simulink model "mimo_2x2_zf"  (R2024b)
settings: Solver=FixedStepDiscrete  StartTime=0  StopTime=0  FixedStep=1  RelTol=1e-3
settings Model: Creator=Devansh  LastModifiedBy=Devansh
settings DataIOCC: SaveOutput=off  SignalLogging=off  SaveTime=off  ReturnWorkspaceOutputs=off

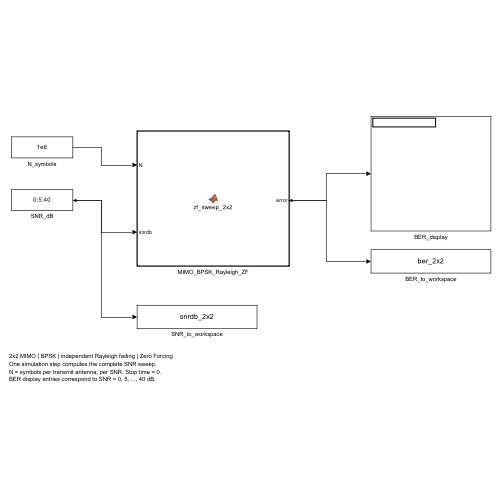
[thumbnail: Simulink's stored preview of the top-level diagram]
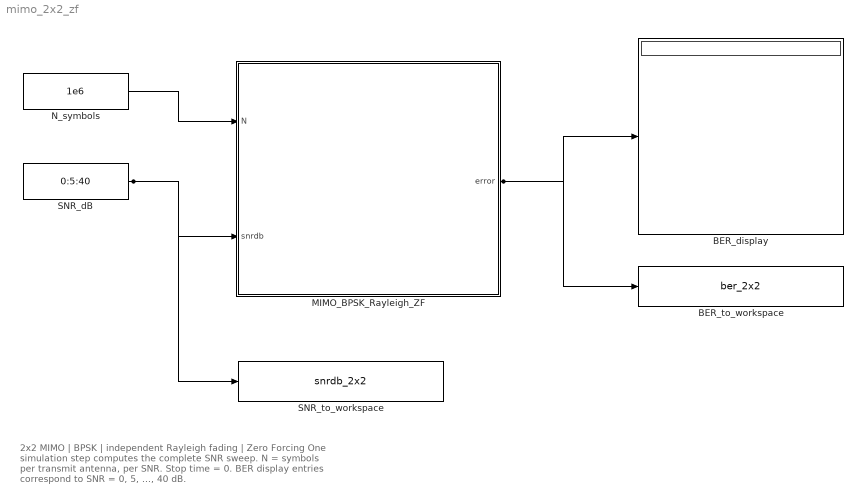
== system mimo_2x2_zf ==
  note: 2x2 MIMO | BPSK | independent Rayleigh fading | Zero Forcing
      | One simulation step computes the complete SNR sweep.
      | N = symbols per transmit antenna, per SNR. Stop time = 0.
      | BER display entries correspond to SNR = 0, 5, ..., 40 dB.
  BER_display : Display
  BER_to_workspace : ToWorkspace  VariableName=ber_2x2  SampleTime=-1
  MIMO_BPSK_Rayleigh_ZF : MATLAB Function  TreatAsAtomicUnit=on
  N_symbols : Constant  Value=1e6  SampleTime=1
  SNR_dB : Constant  Value=0:5:40  SampleTime=1
  SNR_to_workspace : ToWorkspace  VariableName=snrdb_2x2  SampleTime=-1
  wires:
  N_symbols/1 -> MIMO_BPSK_Rayleigh_ZF/1(N)
  SNR_dB/1 -> MIMO_BPSK_Rayleigh_ZF/2(snrdb), SNR_to_workspace/1
  MIMO_BPSK_Rayleigh_ZF/1(error) -> BER_display/1, BER_to_workspace/1

== matlab function mimo_2x2_zf/MIMO_BPSK_Rayleigh_ZF ==
  data: N input; error output; snrdb input
function error = zf_sweep_2x2(N, snrdb)
%#codegen
% Original script calculation; N and snrdb are Constant block inputs.
snrlinear = 10.^(snrdb/10);
nsd = 1 ./ sqrt(snrlinear);
error = zeros(size(snrdb));
for j = 1:length(snrdb)
    x11 = randi(2,1,N)-1;
    x1 = 2*x11-1;
    x22 = randi(2,1,N)-1;
    x2 = 2*x22-1;
    X = [x1;x2];
    h11 = (1/sqrt(2))*complex(randn(1,N),randn(1,N));
    h22 = (1/sqrt(2))*complex(randn(1,N),randn(1,N));
    h12 = (1/sqrt(2))*complex(randn(1,N),randn(1,N));
    h21 = (1/sqrt(2))*complex(randn(1,N),randn(1,N));
    n1 = complex(randn(1,N),randn(1,N))/sqrt(2);
    n2 = complex(randn(1,N),randn(1,N))/sqrt(2);
    y1 = h11.*x1+h12.*x2+n1*nsd(j);
    y2 = h21.*x1+h22.*x2+n2*nsd(j);
    % Explicit complex allocation for MATLAB Function code generation.
    xest = complex(zeros(2,N));
    for i = 1:N
        H = [h11(i),h12(i);h21(i),h22(i)];
        xest(:,i) = H\[y1(i);y2(i)];
    end
    x_detected = 2*(real(xest)>0)-1;
    error(j) = sum(sum(X~=x_detected))/(2*N);
end
end
